simulink model "My_gfm_battery_sil_1_Exciter_Dis"  (R2018b)
settings: Solver=ode23t  StartTime=0.0  StopTime=5  MaxStep=1e-4  RelTol=1e-3
PreLoadFcn:
  | modelDir = fileparts(get_param(bdroot,'FileName'));
  | 
  | load_system(fullfile(modelDir,'controls_element_lib.slx'));
  | load_system(fullfile(modelDir,'test_sequence_lib.slx'));
InitFcn:
  | close all;
  | clear all;
  | clc;
  | 
  | % frequency nominals
  | F_NOM = 60;
  | W_NOM = 2 * pi * F_NOM;
  | 
  | % base values relative to inverter
  | % --------------------------------
  | VLL_INV_NOM = 480;
  | P_INV_NOM = 1e6;
  | Q_INV_NOM = 0.5e6;
  | S_INV_NOM = sqrt(P_INV_NOM^2 + Q_INV_NOM^2);
  | 
  | I_INV_BASE = S_INV_NOM/(sqrt(3)*VLL_INV_NOM);
  | Z_INV_BASE = VLL_INV_NOM^2/S_INV_NOM;
  | L_INV_BASE = Z_INV_BASE / W_NOM;
  | C_INV_BASE = 1 / (Z_INV_BASE * W_NOM);
  | 
  | % nominal ratings for power system model
  | % --------------------------------------
  | INVERTER_COUNT = 100;
  | 
  | VLV_NOM = VLL_INV_NOM;
  | VMV_NOM = 35e3;
  | VHV_NOM = 230e3;
  | S_PLANT = INVERTER_COUNT * S_INV_NOM;
  | 
  | N_GSU = VHV_NOM/VMV_NOM;
  | N_MVT = VMV_NOM/VLV_NOM;
  | 
  | I_LV_BASE = S_PLANT/(sqrt(3)*VLV_NOM);
  | I_MV_BASE = S_PLANT/(sqrt(3)*VMV_NOM);
  | I_HV_BASE = S_PLANT/(sqrt(3)*VHV_NOM);
  | 
  | Z_LV_BASE = VLV_NOM^2/S_PLANT;
  | Z_MV_BASE = VMV_NOM^2/S_PLANT;
  | Z_HV_BASE = VHV_NOM^2/S_PLANT;
  | 
  | L_LV_BASE = Z_LV_BASE / W_NOM;
  | L_MV_BASE = Z_MV_BASE / W_NOM;
  | L_HV_BASE = Z_HV_BASE / W_NOM;
  | C_LV_BASE = 1 / (Z_LV_BASE * W_NOM);
  | C_MV_BASE = 1 / (Z_MV_BASE * W_NOM);
  | C_HV_BASE = 1 / (Z_HV_BASE * W_NOM);
undefined symbols (not defined in the file): D1, D11, Delta, DiscIntNeverNeededParam, gcbh, j, sps_rtmsupport, Ts
libraries: powerlib x70, simulink x29, test_sequence_lib x10, controls_element_lib x3, spsHalfBridgeModel x3
(part 4 of 6)

== system My_gfm_battery_sil_1_Exciter_Dis/My Inverter Controller /My_acMonitor_A/Analyzer_V ==
  note: What is that?
  note: complex multiplication
  note: Let
      | V+*cos wt + V-*cos wt + vo * cos wt + vdc
      | V+*cos (wt-120) + V-*cos (wt+120) vo * cos wt + vdc
      | V+*cos (wt+120) + V-*cos (wt-120) vo * cos wt + vdc
  note: filter to remove pulsating on whatever
      | a frame coming from opposie rotating
  note: + conj
  note: Vd- , Vq-
  note: Vd+ , Vq+
  note: - conj
  note: Not sure why SOGI filter was not used
      | to get clean Pve and Nve
  note: cos x + j sin x
      | cos (x-120) + j (sin x -120)
      | cos (x+120) + j (sin x +120)
  note: cos x - j sin x
  note: V+/2*[1+cos2wt] + V-/2*[1+cos2wt] + vo/2*[1+cos2wt] + vdc * cos wt
      | V+/2*[cos(2pi/3)+cos(2wt-2pi/3)] + V-/2*[cos(2pi/3)+cos(2wt-4pi/3)] + vo/2*[1+cos2wt] + vdc * cos wt
      | V+/2*[cos(2pi/3)+cos(2wt-4pi/3)] + V-/2*[cos(2pi/3)+cos(2wt-2pi/3)] + vo/2*[1+cos2wt] + vdc * cos wt
      |
      | -V+/2*[sin2wt] - V-/2*[sin2wt] - vo/2*[sin2wt] - vdc * sin wt
      | -V+/2*[sin(2wt-2pi/3)+sin(2pi/3)] - V-/2*[sin(2wt-4pi/3)-sin(2pi/3)] - vo/2*[sin2wt] - vdc * sin wt
      | -V+/2*[sin(2wt-4pi/3)-sin(2pi/3)] - V-/2*[sin(2wt-2pi/3)+sin(2pi/3)] - vo/2*[sin2wt] - vdc * sin wt
  note: [ 1 ]
      | [ exp(- j2pi/3)]
      | [ exp(- j4pi/3)]
  note: [ 1 ]
      | [ exp(- j4pi/3)]
      | [ exp(- j8pi/3)] = [ exp(- j2pi/3)]
  note: Remove double frequency
      | V+/2+ V-/2+ vo/2 + vdc*coswt
      | V+/2*cos(2pi/3) + V-/2*cos(2pi/3) + vo/2 + vdc*coswt
      | V+/2*cos(2pi/3) + V-/2*cos(2pi/3) + vo/2 + vdc*coswt
      |
      | - vdc*sinwt
      | -V+/2*sin(2pi/3) - V-/2*-sin(2pi/3) - vdc*sinwt
      | -V+/2*-sin(2pi/3) - V-/2*+sin(2pi/3) - vdc*sinwt
  note: sqrt(2) *[V+/2+ V-/2+ vo/2 + vdc*coswt]
      | sqrt(2) *[V+/2*cos(2pi/3) + V-/2*cos(2pi/3) + vo/2 + vdc*coswt]
      | sqrt(2) *[V+/2*cos(2pi/3) + V-/2*cos(2pi/3) + vo/2 + vdc*coswt]
      |
      | sqrt(2) *[- vdc*sinwt]
      | sqrt(2) *[-V+/2*sin(2pi/3) - V-/2*-sin(2pi/3) - vdc*sinwt]
      | sqrt(2) *[-V+/2*-sin(2pi/3) - V-/2*+sin(2pi/3) - vdc*sinwt]
  note: 1
      | cos(-4pi/3)
      | cos(-2pi/3)
      |
      | 0
      | sin(-4pi/3)
      | sin(-2pi/3)
  note: 1
      | cos(-2pi/3)
      | cos(-4pi/3)
      |
      | 0
      | sin(-2pi/3)
      | sin(-4pi/3)
  note: sqrt(2) *[V+/2+ V-/2+ vo/2 + vdc*coswt] * 1 - sqrt(2) *[- vdc*sinwt] * 0
      | sqrt(2) *[V+/2*cos(2pi/3) + V-/2*cos(2pi/3) + vo/2 + vdc*coswt] * cos(-4pi/3) - sqrt(2) *[-V+/2*sin(2pi/3) - V-/2*-sin(2pi/3) - vdc*sinwt] * sin(-4pi/3)
      | sqrt(2) *[V+/2*cos(2pi/3) + V-/2*cos(2pi/3) + vo/2 + vdc*coswt] * cos(-2pi/3) - sqrt(2) *[-V+/2*-sin(2pi/3) - V-/2*+sin(2pi/3) - vdc*sinwt] * sin(-2pi/3)
      |
      | sqrt(2) *[V+/2+ V-/2+ vo/2 + vdc*coswt] * 0 + sqrt(2) *[- vdc*sinwt] * 1
      | sqrt(2) *[V+/2*cos(2pi/3) + V-/2*cos(2pi/3) + vo/2 + vdc*coswt] * sin(-4pi/3) + sqrt(2) *[-V+/2*sin(2pi/3) - V-/2*-sin(2pi/3) - vdc*sinwt] * cos(-4pi/3)
      | sqrt(2) *[V+/2*cos(2pi/3) + V-/2*cos(2pi/3) + vo/2 + vdc*coswt] * sin(-2pi/3) + sqrt(2) *[-V+/2*-sin(2pi/3) - V-/2*+sin(2pi/3) - vdc*sinwt] * cos(-2pi/3)
  note: 3 * sqrt(2) *[vo/2 + vdc*coswt]
      |
      | 3 * sqrt(2) *[- vdc*sinwt]
  note: sqrt(2) *[vo/2 + vdc*coswt]
      |
      | sqrt(2) *[- vdc*sinwt]
  note: sqrt(2) *[V+/2+ V-/2+ vo/2 + vdc*coswt]
      | sqrt(2) *[V+/2*-0.5 + V-/2*-0.5 + vo/2 + vdc*coswt] * -0.5 - sqrt(2) *[-V+/2*sqrt(3/2) - V-/2*-sqrt(3/2) - vdc*sinwt] * sqrt(3/2)
      | sqrt(2) *[V+/2*-0.5 + V-/2*-0.5 + vo/2 + vdc*coswt] * -0.5 - sqrt(2) *[-V+/2*-sqrt(3/2) - V-/2*+sqrt(3/2) - vdc*sinwt] * -sqrt(3/2)
      |
      | sqrt(2) *[V+/2+ V-/2+ vo/2 + vdc*coswt] * 0 + sqrt(2) *[- vdc*sinwt] * 1
      | sqrt(2) *[V+/2* -0.5 + V-/2* -0.5 + vo/2 + vdc*coswt] * sqrt(3/2) + sqrt(2) *[-V+/2* sqrt(3/2) - V-/2*- sqrt(3/2) - vdc*sinwt] * -0.5
      | sqrt(2) *[V+/2* -0.5 + V-/2* -0.5 + vo/2 + vdc*coswt] * - sqrt(3/2) + sqrt(2) *[-V+/2*- sqrt(3/2) - V-/2* sqrt(3/2) - vdc*sinwt] * -0.5
  note: sqrt(2) *[3 * V+/2+ 0 * V-/2+ 0 * vo/2 + 0 * vdc*coswt
      |
      | sqrt(2) *[0 * V+/2+ 0 * V-/2+ 0 * vo/2 + 0 * vdc*coswt
  note: sqrt(2) *[V+/2]
      |
      | 0
  note: sqrt(3) * sqrt(2) *[V+/2]
      |
      | 0
  note: sqrt(3) *sqrt(2) *[vo/2 + vdc*coswt]
      |
      | sqrt(3)* sqrt(2) *[- vdc*sinwt]
  note: sqrt(2) *[V+/2+ V-/2+ vo/2 + vdc*coswt] * 1 - sqrt(2) *[- vdc*sinwt] * 0
      | sqrt(2) *[V+/2*cos(2pi/3) + V-/2*cos(2pi/3) + vo/2 + vdc*coswt] * cos(-2pi/3) - sqrt(2) *[-V+/2*sin(2pi/3) - V-/2*-sin(2pi/3) - vdc*sinwt] * sin(-2pi/3)
      | sqrt(2) *[V+/2*cos(2pi/3) + V-/2*cos(2pi/3) + vo/2 + vdc*coswt] * cos(-4pi/3) - sqrt(2) *[-V+/2*-sin(2pi/3) - V-/2*+sin(2pi/3) - vdc*sinwt] * sin(-4pi/3)
      |
      | sqrt(2) *[V+/2+ V-/2+ vo/2 + vdc*coswt] * 0 + sqrt(2) *[- vdc*sinwt] * 1
      | sqrt(2) *[V+/2*cos(2pi/3) + V-/2*cos(2pi/3) + vo/2 + vdc*coswt] * sin(-2pi/3) + sqrt(2) *[-V+/2*sin(2pi/3) - V-/2*-sin(2pi/3) - vdc*sinwt] * cos(-2pi/3)
      | sqrt(2) *[V+/2*cos(2pi/3) + V-/2*cos(2pi/3) + vo/2 + vdc*coswt] * sin(-4pi/3) + sqrt(2) *[-V+/2*-sin(2pi/3) - V-/2*+sin(2pi/3) - vdc*sinwt] * cos(-4pi/3)
  note: sqrt(2) *[V+/2+ V-/2+ vo/2 + vdc*coswt]
      | sqrt(2) *[V+/2*-0.5 + V-/2*-0.5 + vo/2 + vdc*coswt] * -0.5 - sqrt(2) *[-V+/2*sqrt(3/2) - V-/2*-sqrt(3/2) - vdc*sinwt] * -sqrt(3/2)
      | sqrt(2) *[V+/2*-0.5 + V-/2*-0.5 + vo/2 + vdc*coswt] * -0.5 - sqrt(2) *[-V+/2*-sqrt(3/2) - V-/2*+sqrt(3/2) - vdc*sinwt] * sqrt(3/2)
      |
      | sqrt(2) *[V+/2+ V-/2+ vo/2 + vdc*coswt] * 0 + sqrt(2) *[- vdc*sinwt] * 1
      | sqrt(2) *[V+/2*-0.5 + V-/2*-0.5 + vo/2 + vdc*coswt] * -sqrt(3/2) + sqrt(2) *[-V+/2*sqrt(3/2) - V-/2*-sqrt(3/2) - vdc*sinwt] * -0.5
      | sqrt(2) *[V+/2*-0.5 + V-/2*-0.5 + vo/2 + vdc*coswt] * sqrt(3/2) + sqrt(2) *[-V+/2*-sqrt(3/2) - V-/2*sqrt(3/2) - vdc*sinwt] * -0.5
  note: sqrt(2) *[0 * V+/2+ 3 * V-/2+ 0 * vo/2 + 0 * vdc*coswt
      |
      | sqrt(2) *[0 * V+/2+ 0 * V-/2+ 0 * vo/2 + 0 * vdc*coswt
  note: sqrt(2) *[V-/2]
      |
      | 0
  note: sqrt(3) *sqrt(2) *[V-/2]
      |
      | 0
  note: sqrt(2) *[V+/2+ V-/2+ vo/2 + vdc*coswt]
      | sqrt(2) *[V+/2*cos(2pi/3) + V-/2*cos(2pi/3) + vo/2 + vdc*coswt] * cos(-4pi/3) - sqrt(2) *[-V+/2*sin(2pi/3) - V-/2*-sin(2pi/3) - vdc*sinwt] * sin(-4pi/3)
      | sqrt(2) *[V+/2*cos(2pi/3) + V-/2*cos(2pi/3) + vo/2 + vdc*coswt] * cos(-2pi/3) - sqrt(2) *[-V+/2*-sin(2pi/3) - V-/2*+sin(2pi/3) - vdc*sinwt] * sin(-2pi/3)
      |
      | sqrt(2) *[- vdc*sinwt]
      | sqrt(2) *[V+/2*cos(2pi/3) + V-/2*cos(2pi/3) + vo/2 + vdc*coswt] * sin(-4pi/3) + sqrt(2) *[-V+/2*sin(2pi/3) - V-/2*-sin(2pi/3) - vdc*sinwt] * cos(-4pi/3)
      | sqrt(2) *[V+/2*cos(2pi/3) + V-/2*cos(2pi/3) + vo/2 + vdc*coswt] * sin(-2pi/3) + sqrt(2) *[-V+/2*-sin(2pi/3) - V-/2*+sin(2pi/3) - vdc*sinwt] * cos(-2pi/3)
  in[3] : Inport
  osc[3] : Inport  Port=2
  Conj : Math  Operator=conj  SaturateOnIntegerOverflow=on
  Demux : Demux  Outputs=3
  Gain2 : Gain  Gain=1/3
  Gain3 : Gain  Gain=1/3
  Gain4 : Gain  Gain=1/3
  Gain5 : Gain  Gain=sqrt(2)
  Product1 : Product
  Product2 : Product
  Product3 : Product
  Rotation : Constant  Value=exp(j*2*pi*[0 -1/3 -2/3])
  Rotation1 : Constant  Value=exp(j*2*pi*[0 -1/3 -2/3])
  Square : Math  Operator=square  SaturateOnIntegerOverflow=on
  Sum of Elements1 : Sum  Inputs=+
  Sum of Elements2 : Sum  Inputs=+
  Sum of Elements3 : Sum  Inputs=+
  Terminator : Terminator
  Terminator1 : Terminator
  complex_LPF : Subsystem  mask{tau=0.05}
      mask prompts: tau "Time constant"
  convert_to_LL : Gain  Gain=sqrt(3)
  convert_to_LL1 : Gain  Gain=sqrt(3)
  convert_to_LL2 : Gain  Gain=sqrt(3)
  fund[3] : Outport  VectorParamsAs1DForOutWhenUnconnected=on
  Zero : Outport  Port=2  VectorParamsAs1DForOutWhenUnconnected=on
  Pve : Outport  Port=3  VectorParamsAs1DForOutWhenUnconnected=on
  Nve : Outport  Port=4  VectorParamsAs1DForOutWhenUnconnected=on
  wires:
  convert_to_LL2/1 -> Nve/1
  convert_to_LL1/1 -> Pve/1
  convert_to_LL/1 -> Zero/1
  Gain4/1 -> convert_to_LL2/1
  complex_LPF/1(Out1) -> Gain5/1
  Product3/1 -> Sum of Elements3/1
  Product1/1 -> complex_LPF/1(In1)
  Demux/1 -> Conj/1
  Rotation/1 -> Square/1
  Rotation1/1 -> Product3/2
  Sum of Elements2/1 -> Gain3/1
  Conj/1 -> Product1/2
  Sum of Elements1/1 -> Gain2/1
  Square/1 -> Product2/2
  Sum of Elements3/1 -> Gain4/1
  osc[3]/1 -> Demux/1
  Gain3/1 -> convert_to_LL1/1
  Gain2/1 -> convert_to_LL/1
  in[3]/1 -> Product1/1
  Demux/2 -> Terminator/1
  Demux/3 -> Terminator1/1
  Gain5/1 -> Sum of Elements1/1, Product3/1, Product2/1
  Product2/1 -> Sum of Elements2/1, fund[3]/1

== system My_gfm_battery_sil_1_Exciter_Dis/My Inverter Controller /My_acMonitor_A/Analyzer_V1 ==
  note: Let Va coswt, so
      | V/2 *[ exp(jw) +exp(-jw)]
      | V/2 *[ exp(jw - j2pi/3) +exp(-jw + j2pi/3)]
      | V/2 *[ exp(jw - j4pi/3) +exp(-jw + j4pi/3)]
  note: filter to remove pulsating on whatever
      | a frame coming from opposie rotating
  note: + conj
  note: Vd- , Vq-
  note: Vd+ , Vq+
  note: - conj
  note: Not sure why SOGI filter was not used
      | to get clean Pve and Nve
  note: cos x + j sin x
      | cos (x-120) + j (sin x -120)
      | cos (x+120) + j (sin x +120)
  note: cos x - j sin x
  note: V/2 *[ 1 +exp(-2jw)]
      | V/2 *[ exp(- j2pi/3) +exp(-2jw + j2pi/3)]
      | V/2 *[ exp(- j4pi/3) +exp(-2jw + j4pi/3)]
  note: Remove double frequency
      | V/2 *[ 1 ]
      | V/2 *[ exp(- j2pi/3)]
      | V/2 *[ exp(- j4pi/3)]
  note: sqrt(2) * V/2 *[ 1 ]
      | sqrt(2) * V/2 *[ exp(- j2pi/3)]
      | sqrt(2) * V/2 *[ exp(- j4pi/3)]
  note: [ 1 ]
      | [ exp(- j2pi/3)]
      | [ exp(- j4pi/3)]
  note: sqrt(2) * V/2 *[ 1 ]
      | sqrt(2) * V/2 *[ exp(- j4pi/3)]
      | sqrt(2) * V/2 *[ exp(- j8pi/3)] = sqrt(2) * V/2 *[ exp(- j2pi/3)]
  note: [ 1 ]
      | [ exp(- j4pi/3)]
      | [ exp(- j8pi/3)] = [ exp(- j2pi/3)]
  note: sqrt(2) * V/2 *[ 1 ]
      | sqrt(2) * V/2 *[ exp(- j6pi/3)] = sqrt(2) * Vb/2
      | sqrt(2) * V/2 *[ exp(- j6pi/3)] = sqrt(2) * Vc/2
  note: sqrt(2) * V/2 *[ 1 ]
      | + sqrt(2) * V/2 *[ exp(- j2pi/3)]
      | + sqrt(2) * V/2 *[ exp(- j4pi/3)]
      | = 0
  note: sqrt(2) * V/2
      | + sqrt(2) * V/2
      | + sqrt(2) * V/2
      | = 3 * sqrt(2) * V/2 * 1/3 = V/sqrt(2)
      | The LN RMS
  note: sqrt(2) * V/2
      | + sqrt(2) * V/2 *[ exp(- j4pi/3)]
      | + sqrt(2) * V/2 *[ exp(- j2pi/3)]
      | = 0
      | The LN RMS
  in[3] : Inport
  osc[3] : Inport  Port=2
  Conj : Math  Operator=conj  SaturateOnIntegerOverflow=on
  Demux : Demux  Outputs=3
  Gain2 : Gain  Gain=1/3
  Gain3 : Gain  Gain=1/3
  Gain4 : Gain  Gain=1/3
  Gain5 : Gain  Gain=sqrt(2)
  Product1 : Product
  Product2 : Product
  Product3 : Product
  Rotation : Constant  Value=exp(j*2*pi*[0 -1/3 -2/3])
  Rotation1 : Constant  Value=exp(j*2*pi*[0 -1/3 -2/3])
  Square : Math  Operator=square  SaturateOnIntegerOverflow=on
  Sum of Elements1 : Sum  Inputs=+
  Sum of Elements2 : Sum  Inputs=+
  Sum of Elements3 : Sum  Inputs=+
  Terminator : Terminator
  Terminator1 : Terminator
  complex_LPF : Subsystem  mask{tau=0.05}
      mask prompts: tau "Time constant"
  convert_to_LL : Gain  Gain=sqrt(3)
  convert_to_LL1 : Gain  Gain=sqrt(3)
  convert_to_LL2 : Gain  Gain=sqrt(3)
  fund[3] : Outport  VectorParamsAs1DForOutWhenUnconnected=on
  Zero : Outport  Port=2  VectorParamsAs1DForOutWhenUnconnected=on
  Pve : Outport  Port=3  VectorParamsAs1DForOutWhenUnconnected=on
  Nve : Outport  Port=4  VectorParamsAs1DForOutWhenUnconnected=on
  wires:
  convert_to_LL2/1 -> Nve/1
  convert_to_LL1/1 -> Pve/1
  convert_to_LL/1 -> Zero/1
  Gain4/1 -> convert_to_LL2/1
  Product2/1 -> fund[3]/1, Sum of Elements2/1
  complex_LPF/1(Out1) -> Gain5/1
  Product3/1 -> Sum of Elements3/1
  Product1/1 -> complex_LPF/1(In1)
  Demux/1 -> Conj/1
  Rotation/1 -> Square/1
  Rotation1/1 -> Product3/2
  Sum of Elements2/1 -> Gain3/1
  Conj/1 -> Product1/2
  Sum of Elements1/1 -> Gain2/1
  Square/1 -> Product2/2
  Sum of Elements3/1 -> Gain4/1
  osc[3]/1 -> Demux/1
  Gain3/1 -> convert_to_LL1/1
  Gain2/1 -> convert_to_LL/1
  in[3]/1 -> Product1/1
  Demux/2 -> Terminator/1
  Demux/3 -> Terminator1/1
  Gain5/1 -> Sum of Elements1/1, Product3/1, Product2/1

== system My_gfm_battery_sil_1_Exciter_Dis/My Inverter Controller /My_acMonitor_A/PLL_3ph ==
  note: cos x - j sin x
      | cos (x-120) - j (sin x -120)
      | cos (x+120) - j (sin x +120)
  note: cos x + j sin x
      | cos (x-120) + j (sin x -120)
      | cos (x+120) + j (sin x +120)
  note: -sin x
      |  -sin (x -120)
      |  -sin (x +120)
  note: Vq
  note: filter 120 Hz, due to negative sequence
  note: Leaky Integrator
  note: vd = Va * cos x + Vb * cos (x-120) + Vc * cos (x+120)
  note: vq = -Va * sin x - Vb * sin (x-120) - Vc * sin (x+120)
  note: Va = vd * cos x - vq * sin x
  note: Vb = vd * cos (x-120) - vq * sin (x-120)
  note: Vc = vd * cos (x+120) - vq * sin (x+120)
  ref : Inport
  Complex to Real-Imag : ComplexToRealImag
  Conj : Math  Operator=conj  SaturateOnIntegerOverflow=on
  Constant : Constant  Value=120
  Gain1 : Gain  Gain=1.5
  Gain2 : Gain  Gain=4.5
  Gain3 : Gain  Gain=10e-3
  Integrator : Integrator  LimitOutput=on  UpperSaturationLimit=5  LowerSaturationLimit=-5
  Product : Product
  SOGI : controls_element_lib/dcVoltageRegulator_A/SOGI  SystemSampleTime=-1
  Saturation : Saturate  UpperLimit=5  LowerLimit=-5
  Sum : Sum  Inputs=+++
  Sum of Elements : Sum  Inputs=+
  Sum1 : Sum  Inputs=|+-
  Terminator : Terminator
  Terminator1 : Terminator
  Transfer Fcn : TransferFcn  Denominator=[0.02 1]
  f_nom : Constant  Value=nominalFrequency
  oscillator_3ph : Subsystem
  osc[3] : Outport  VectorParamsAs1DForOutWhenUnconnected=on
  freq : Outport  Port=2  VectorParamsAs1DForOutWhenUnconnected=on
  wires:
  Constant/1 -> SOGI/2
  Transfer Fcn/1 -> SOGI/1  "phase_error"
  f_nom/1 -> Sum/1
  Gain3/1 -> Sum1/2
  Sum of Elements/1 -> Transfer Fcn/1
  SOGI/1 -> Gain1/1, Gain2/1  "phase_error"
  Saturation/1 -> Sum/2
  Product/1 -> Sum of Elements/1
  Sum/1 -> freq/1, oscillator_3ph/1(f)  "freq"
  oscillator_3ph/1(osc[3]) -> Conj/1, osc[3]/1
  Gain2/1 -> Sum1/1
  Complex to Real-Imag/2 -> Product/2
  Sum1/1 -> Integrator/1
  Integrator/1 -> Gain3/1, Sum/3
  ref/1 -> Product/1
  Conj/1 -> Complex to Real-Imag/1
  Gain1/1 -> Saturation/1
  Complex to Real-Imag/1 -> Terminator/1
  SOGI/2 -> Terminator1/1

== system My_gfm_battery_sil_1_Exciter_Dis/My Inverter Controller /My_acMonitor_A/RMS_Analyzer ==
  in : Inport
  Gain : Gain  Gain=2 * pi * 10
  Integrator : Integrator  InitialCondition=0.01
  Sqrt : Sqrt  SaturateOnIntegerOverflow=on
  Square : Math  Operator=square  SaturateOnIntegerOverflow=on
  Sum : Sum  Inputs=|+-
  RMS : Outport  VectorParamsAs1DForOutWhenUnconnected=on
  wires:
  Square/1 -> Sum/1
  in/1 -> Square/1
  Gain/1 -> Integrator/1
  Sum/1 -> Gain/1
  Integrator/1 -> Sum/2, Sqrt/1
  Sqrt/1 -> RMS/1

== system My_gfm_battery_sil_1_Exciter_Dis/My Inverter Controller /My_acMonitor_A/SOGI ==
  in : Inport
  fnom : Inport  Port=2
  2pi : Gain  Gain=2*pi
  Integrator2 : Integrator
  Integrator3 : Integrator
  Product : Product
  Product1 : Product
  Sum4 : Sum  Inputs=|+-
  Sum5 : Sum  Inputs=|+-
  alpha : Gain  Gain=1 / sqrt(2)
  notch : Outport  VectorParamsAs1DForOutWhenUnconnected=on
  bpf : Outport  Port=2  VectorParamsAs1DForOutWhenUnconnected=on
  wires:
  Product1/1 -> Integrator3/1
  Product/1 -> Integrator2/1
  2pi/1 -> Product/2, Product1/2
  Integrator3/1 -> Sum4/2
  Sum4/1 -> Product/1
  Sum5/1 -> notch/1, alpha/1
  alpha/1 -> Sum4/1
  Integrator2/1 -> bpf/1, Sum5/2, Product1/1
  fnom/1 -> 2pi/1
  in/1 -> Sum5/1

== system My_gfm_battery_sil_1_Exciter_Dis/My Inverter Controller /My_circuit_controls_A/LPF1 ==
  note: Forward integrator
  in : Inport
  Constant2 : Constant  Value=Ts
  Constant3 : Constant  Value=OmegaUp
  Constant4 : Constant  Value=OmegaDn
  Constant9 : Constant  Value=1/20000
  Delay : Delay  DelayLength=1  InitialCondition=0
  Gain : Gain  Gain=1/5
  Math Function : Math  Operator=reciprocal  SaturateOnIntegerOverflow=on
  MinMax : MinMax  Function=max  Inputs=2
  MinMax1 : MinMax  Inputs=2
  MinMax2 : MinMax  Inputs=2
  Product : Product
  Product1 : Product
  Product2 : Product
  Saturation : Saturate  UpperLimit=inf  LowerLimit=0
  Saturation1 : Saturate  UpperLimit=0  LowerLimit=-inf
  Sum : Sum  Inputs=|++
  Sum1 : Sum  Inputs=|++
  Sum4 : Sum  Inputs=|+-
  out : Outport  VectorParamsAs1DForOutWhenUnconnected=on
  wires:
  Delay/1 -> out/1, Sum4/2, Sum/2
  in/1 -> Sum4/1
  Sum4/1 -> Product2/1, Product1/2
  Sum/1 -> Delay/1
  Saturation/1 -> Sum1/1
  Saturation1/1 -> Sum1/2
  Sum1/1 -> Product/2
  Product/1 -> Sum/1
  [Ts] -> Product/1
  [OmegaUp] -> Product1/1
  [OmegaDn] -> Product2/2
  Constant2/1 -> MinMax/1
  MinMax/1 -> [Ts]
  Constant9/1 -> MinMax/2
  MinMax1/1 -> [OmegaUp]
  MinMax2/1 -> [OmegaDn]
  [Ts] -> Math Function/1
  Math Function/1 -> Gain/1
  Gain/1 -> MinMax1/2, MinMax2/1
  Constant3/1 -> MinMax1/1
  Constant4/1 -> MinMax2/2
  Product1/1 -> Saturation/1
  Product2/1 -> Saturation1/1

== system My_gfm_battery_sil_1_Exciter_Dis/My Inverter Controller /My_circuit_controls_A/LPF2 ==
  note: Forward integrator
  in : Inport
  Constant2 : Constant  Value=Ts
  Constant3 : Constant  Value=OmegaUp
  Constant4 : Constant  Value=OmegaDn
  Constant9 : Constant  Value=1/20000
  Delay : Delay  DelayLength=1  InitialCondition=0
  Gain : Gain  Gain=1/5
  Math Function : Math  Operator=reciprocal  SaturateOnIntegerOverflow=on
  MinMax : MinMax  Function=max  Inputs=2
  MinMax1 : MinMax  Inputs=2
  MinMax2 : MinMax  Inputs=2
  Product : Product
  Product1 : Product
  Product2 : Product
  Saturation : Saturate  UpperLimit=inf  LowerLimit=0
  Saturation1 : Saturate  UpperLimit=0  LowerLimit=-inf
  Sum : Sum  Inputs=|++
  Sum1 : Sum  Inputs=|++
  Sum4 : Sum  Inputs=|+-
  out : Outport  VectorParamsAs1DForOutWhenUnconnected=on
  wires:
  Delay/1 -> out/1, Sum4/2, Sum/2
  in/1 -> Sum4/1
  Sum4/1 -> Product2/1, Product1/2
  Sum/1 -> Delay/1
  Saturation/1 -> Sum1/1
  Saturation1/1 -> Sum1/2
  Sum1/1 -> Product/2
  Product/1 -> Sum/1
  [Ts] -> Product/1
  [OmegaUp] -> Product1/1
  [OmegaDn] -> Product2/2
  Constant2/1 -> MinMax/1
  MinMax/1 -> [Ts]
  Constant9/1 -> MinMax/2
  MinMax1/1 -> [OmegaUp]
  MinMax2/1 -> [OmegaDn]
  [Ts] -> Math Function/1
  Math Function/1 -> Gain/1
  Gain/1 -> MinMax1/2, MinMax2/1
  Constant3/1 -> MinMax1/1
  Constant4/1 -> MinMax2/2
  Product1/1 -> Saturation/1
  Product2/1 -> Saturation1/1

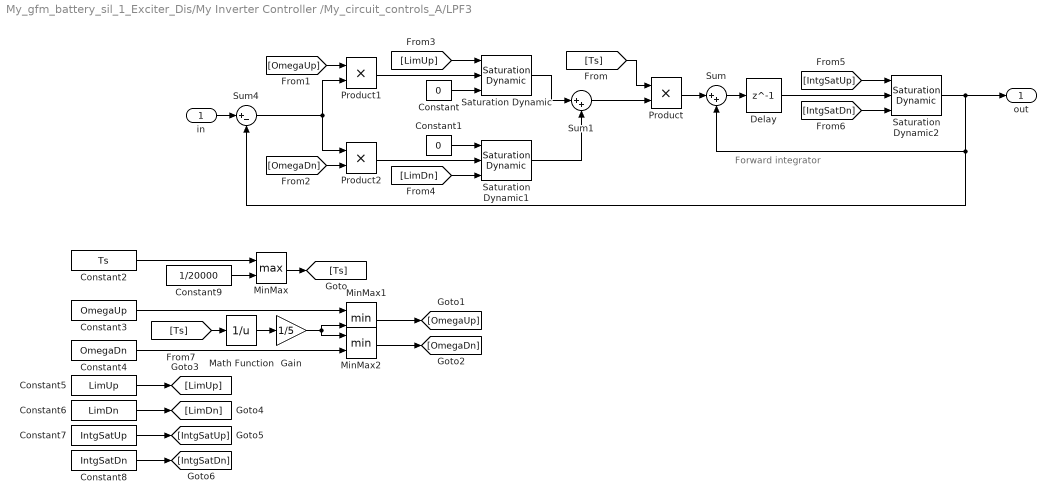
== system My_gfm_battery_sil_1_Exciter_Dis/My Inverter Controller /My_circuit_controls_A/LPF3 ==
  note: Forward integrator
  in : Inport
  Constant : Constant  Value=0
  Constant1 : Constant  Value=0
  Constant2 : Constant  Value=Ts
  Constant3 : Constant  Value=OmegaUp
  Constant4 : Constant  Value=OmegaDn
  Constant5 : Constant  Value=LimUp
  Constant6 : Constant  Value=LimDn
  Constant7 : Constant  Value=IntgSatUp
  Constant8 : Constant  Value=IntgSatDn
  Constant9 : Constant  Value=1/20000
  Delay : Delay  DelayLength=1  InitialCondition=0
  Gain : Gain  Gain=1/5
  Math Function : Math  Operator=reciprocal  SaturateOnIntegerOverflow=on
  MinMax : MinMax  Function=max  Inputs=2
  MinMax1 : MinMax  Inputs=2
  MinMax2 : MinMax  Inputs=2
  Product : Product
  Product1 : Product
  Product2 : Product
  Saturation Dynamic : simulink/Discontinuities/Saturation Dynamic  OutMin=[]  OutMax=[]  OutDataTypeStr=Inherit: Same as second input  OutDataType=fixdt(1, 16)  OutScaling=2^-10  DoSatur=off
  Saturation Dynamic1 : simulink/Discontinuities/Saturation Dynamic  OutMin=[]  OutMax=[]  OutDataTypeStr=Inherit: Same as second input  OutDataType=fixdt(1, 16)  OutScaling=2^-10  DoSatur=off
  Saturation Dynamic2 : simulink/Discontinuities/Saturation Dynamic  OutMin=[]  OutMax=[]  OutDataTypeStr=Inherit: Same as second input  OutDataType=fixdt(1, 16)  OutScaling=2^-10  DoSatur=off
  Sum : Sum  Inputs=|++
  Sum1 : Sum  Inputs=|++
  Sum4 : Sum  Inputs=|+-
  out : Outport  VectorParamsAs1DForOutWhenUnconnected=on
  wires:
  Saturation Dynamic2/1 -> Sum/2, Sum4/2, out/1
  in/1 -> Sum4/1
  Sum4/1 -> Product2/1, Product1/2
  Product1/1 -> Saturation Dynamic/2
  Product2/1 -> Saturation Dynamic1/2
  Sum/1 -> Delay/1
  Delay/1 -> Saturation Dynamic2/2
  Saturation Dynamic/1 -> Sum1/1
  Saturation Dynamic1/1 -> Sum1/2
  Sum1/1 -> Product/2
  Product/1 -> Sum/1
  [Ts] -> Product/1
  [OmegaUp] -> Product1/1
  [OmegaDn] -> Product2/2
  Constant/1 -> Saturation Dynamic/3
  Constant1/1 -> Saturation Dynamic1/1
  [LimUp] -> Saturation Dynamic/1
  [LimDn] -> Saturation Dynamic1/3
  Constant2/1 -> MinMax/1
  Constant5/1 -> [LimUp]
  Constant6/1 -> [LimDn]
  [IntgSatUp] -> Saturation Dynamic2/1
  [IntgSatDn] -> Saturation Dynamic2/3
  Constant7/1 -> [IntgSatUp]
  Constant8/1 -> [IntgSatDn]
  MinMax/1 -> [Ts]
  Constant9/1 -> MinMax/2
  MinMax1/1 -> [OmegaUp]
  MinMax2/1 -> [OmegaDn]
  [Ts] -> Math Function/1
  Math Function/1 -> Gain/1
  Gain/1 -> MinMax1/2, MinMax2/1
  Constant3/1 -> MinMax1/1
  Constant4/1 -> MinMax2/2

== system My_gfm_battery_sil_1_Exciter_Dis/My Inverter Controller /My_circuit_controls_A/LPF4 ==
  note: Forward integrator
  in : Inport
  Constant2 : Constant  Value=Ts
  Constant3 : Constant  Value=OmegaUp
  Constant4 : Constant  Value=OmegaDn
  Constant9 : Constant  Value=1/20000
  Delay : Delay  DelayLength=1  InitialCondition=0
  Gain : Gain  Gain=1/5
  Math Function : Math  Operator=reciprocal  SaturateOnIntegerOverflow=on
  MinMax : MinMax  Function=max  Inputs=2
  MinMax1 : MinMax  Inputs=2
  MinMax2 : MinMax  Inputs=2
  Product : Product
  Product1 : Product
  Product2 : Product
  Saturation : Saturate  UpperLimit=inf  LowerLimit=0
  Saturation1 : Saturate  UpperLimit=0  LowerLimit=-inf
  Sum : Sum  Inputs=|++
  Sum1 : Sum  Inputs=|++
  Sum4 : Sum  Inputs=|+-
  out : Outport  VectorParamsAs1DForOutWhenUnconnected=on
  wires:
  Delay/1 -> out/1, Sum4/2, Sum/2
  in/1 -> Sum4/1
  Sum4/1 -> Product2/1, Product1/2
  Sum/1 -> Delay/1
  Saturation/1 -> Sum1/1
  Saturation1/1 -> Sum1/2
  Sum1/1 -> Product/2
  Product/1 -> Sum/1
  [Ts] -> Product/1
  [OmegaUp] -> Product1/1
  [OmegaDn] -> Product2/2
  Constant2/1 -> MinMax/1
  MinMax/1 -> [Ts]
  Constant9/1 -> MinMax/2
  MinMax1/1 -> [OmegaUp]
  MinMax2/1 -> [OmegaDn]
  [Ts] -> Math Function/1
  Math Function/1 -> Gain/1
  Gain/1 -> MinMax1/2, MinMax2/1
  Constant3/1 -> MinMax1/1
  Constant4/1 -> MinMax2/2
  Product1/1 -> Saturation/1
  Product2/1 -> Saturation1/1

== system My_gfm_battery_sil_1_Exciter_Dis/My Inverter Controller /My_circuit_controls_A/LPF5 ==
  note: Forward integrator
  in : Inport
  Constant2 : Constant  Value=Ts
  Constant3 : Constant  Value=OmegaUp
  Constant4 : Constant  Value=OmegaDn
  Constant9 : Constant  Value=1/20000
  Delay : Delay  DelayLength=1  InitialCondition=0
  Gain : Gain  Gain=1/5
  Math Function : Math  Operator=reciprocal  SaturateOnIntegerOverflow=on
  MinMax : MinMax  Function=max  Inputs=2
  MinMax1 : MinMax  Inputs=2
  MinMax2 : MinMax  Inputs=2
  Product : Product
  Product1 : Product
  Product2 : Product
  Saturation : Saturate  UpperLimit=inf  LowerLimit=0
  Saturation1 : Saturate  UpperLimit=0  LowerLimit=-inf
  Sum : Sum  Inputs=|++
  Sum1 : Sum  Inputs=|++
  Sum4 : Sum  Inputs=|+-
  out : Outport  VectorParamsAs1DForOutWhenUnconnected=on
  wires:
  Delay/1 -> out/1, Sum4/2, Sum/2
  in/1 -> Sum4/1
  Sum4/1 -> Product2/1, Product1/2
  Sum/1 -> Delay/1
  Saturation/1 -> Sum1/1
  Saturation1/1 -> Sum1/2
  Sum1/1 -> Product/2
  Product/1 -> Sum/1
  [Ts] -> Product/1
  [OmegaUp] -> Product1/1
  [OmegaDn] -> Product2/2
  Constant2/1 -> MinMax/1
  MinMax/1 -> [Ts]
  Constant9/1 -> MinMax/2
  MinMax1/1 -> [OmegaUp]
  MinMax2/1 -> [OmegaDn]
  [Ts] -> Math Function/1
  Math Function/1 -> Gain/1
  Gain/1 -> MinMax1/2, MinMax2/1
  Constant3/1 -> MinMax1/1
  Constant4/1 -> MinMax2/2
  Product1/1 -> Saturation/1
  Product2/1 -> Saturation1/1

== system My_gfm_battery_sil_1_Exciter_Dis/My Inverter Controller /My_circuit_controls_A/SOGI ==
  in : Inport
  f : Inport  Port=2
  Constant2 : Constant  Value=Ts
  Constant9 : Constant  Value=1/20000
  Gain : Gain
  Gain2 : Gain  Gain=2*pi
  Integrator1 : Subsystem
  Integrator3 : Subsystem
  MinMax : MinMax  Function=max  Inputs=2
  Product : Product
  Product2 : Product
  Sum : Sum  Inputs=|+-
  Sum1 : Sum  Inputs=|+-
  Notched : Outport  VectorParamsAs1DForOutWhenUnconnected=on
  BandPassed : Outport  Port=2  VectorParamsAs1DForOutWhenUnconnected=on
  wires:
  f/1 -> Gain2/1
  in/1 -> Sum1/1
  Integrator1/1(Out) -> Product2/1
  Gain/1 -> Sum1/2
  Sum1/1 -> Notched/1, Sum/1
  Integrator3/1(Out) -> Gain/1, BandPassed/1, Integrator1/1(In)
  Gain2/1 -> Product2/2, Product/2
  Sum/1 -> Product/1
  Product2/1 -> Sum/2
  [Ts] -> Integrator3/2(Ts)
  Product/1 -> Integrator3/1(In)
  [Ts] -> Integrator1/2(Ts)
  MinMax/1 -> [Ts]
  Constant2/1 -> MinMax/1
  Constant9/1 -> MinMax/2

== system My_gfm_battery_sil_1_Exciter_Dis/My Inverter Controller /My_circuit_controls_A/SOGI_BPF1 ==
  in : Inport
  f : Inport  Port=2
  Gain : Gain
  Gain2 : Gain  Gain=2*pi
  Integrator : Integrator
  Integrator1 : Integrator
  Product : Product
  Product2 : Product
  Sum : Sum  Inputs=|+-
  Sum1 : Sum  Inputs=|+-
  Notched : Outport  VectorParamsAs1DForOutWhenUnconnected=on
  BandPassed : Outport  Port=2  VectorParamsAs1DForOutWhenUnconnected=on
  wires:
  f/1 -> Gain2/1
  in/1 -> Sum1/1
  Product/1 -> Integrator/1
  Integrator1/1 -> Product2/1
  Gain/1 -> Sum1/2
  Sum1/1 -> Notched/1, Sum/1
  Integrator/1 -> BandPassed/1, Integrator1/1, Gain/1
  Gain2/1 -> Product2/2, Product/2
  Sum/1 -> Product/1
  Product2/1 -> Sum/2

== system My_gfm_battery_sil_1_Exciter_Dis/My Inverter Controller /My_circuit_controls_A/virtual damper ==
  v : Inport
  Damping HPF : Subsystem  mask(High Pass Filter){Ts=1/20000, OmegaUp=1/250e-6, OmegaDn=1/250e-6}
      mask prompts: Ts "Tsample"; OmegaUp "Up Path Bandwidth"; OmegaDn "Down Path Bandwidth"
      mask help: Min. Tsample is 1/20000; Max. Omega is 0.2/Ts
      mask DialogControl Container2 Prompt: Parameters
  g_damp : Gain  Gain=1/(0.8*Z_INV_BASE)
  i_damp : Outport  VectorParamsAs1DForOutWhenUnconnected=on
  wires:
  g_damp/1 -> i_damp/1
  v/1 -> Damping HPF/1(in)
  Damping HPF/1(out) -> g_damp/1

== system My_gfm_battery_sil_1_Exciter_Dis/My Inverter Controller /My_circuit_controls_A/virtual damper1 ==
  v : Inport
  1/tau_damp : Gain  Gain=1/250e-6
  Integrator : Integrator
  Sum : Sum  Inputs=|+-
  g_damp : Gain  Gain=1/(0.8*Z_INV_BASE)
  i_damp : Outport  VectorParamsAs1DForOutWhenUnconnected=on
  wires:
  g_damp/1 -> i_damp/1
  Sum/1 -> g_damp/1, 1/tau_damp/1
  v/1 -> Sum/1
  1/tau_damp/1 -> Integrator/1
  Integrator/1 -> Sum/2

== system My_gfm_battery_sil_1_Exciter_Dis/My Inverter Controller /My_circuit_controls_A1/LPF ==
  1 : Inport
  Gain2 : Gain  Gain=1/20e-6
  Integrator : Integrator
  Sum4 : Sum  Inputs=|+-
  Out1 : Outport  VectorParamsAs1DForOutWhenUnconnected=on
  wires:
  Gain2/1 -> Integrator/1
  Integrator/1 -> Sum4/2, Out1/1
  1/1 -> Sum4/1
  Sum4/1 -> Gain2/1

== system My_gfm_battery_sil_1_Exciter_Dis/My Inverter Controller /My_circuit_controls_A1/LPF1 ==
  note: Forward integrator
  in : Inport
  Constant2 : Constant  Value=Ts
  Constant3 : Constant  Value=OmegaUp
  Constant4 : Constant  Value=OmegaDn
  Constant9 : Constant  Value=1/20000
  Delay : Delay  DelayLength=1  InitialCondition=0
  Gain : Gain  Gain=1/5
  Math Function : Math  Operator=reciprocal  SaturateOnIntegerOverflow=on
  MinMax : MinMax  Function=max  Inputs=2
  MinMax1 : MinMax  Inputs=2
  MinMax2 : MinMax  Inputs=2
  Product : Product
  Product1 : Product
  Product2 : Product
  Saturation : Saturate  UpperLimit=inf  LowerLimit=0
  Saturation1 : Saturate  UpperLimit=0  LowerLimit=-inf
  Sum : Sum  Inputs=|++
  Sum1 : Sum  Inputs=|++
  Sum4 : Sum  Inputs=|+-
  out : Outport  VectorParamsAs1DForOutWhenUnconnected=on
  wires:
  Delay/1 -> out/1, Sum4/2, Sum/2
  in/1 -> Sum4/1
  Sum4/1 -> Product2/1, Product1/2
  Sum/1 -> Delay/1
  Saturation/1 -> Sum1/1
  Saturation1/1 -> Sum1/2
  Sum1/1 -> Product/2
  Product/1 -> Sum/1
  [Ts] -> Product/1
  [OmegaUp] -> Product1/1
  [OmegaDn] -> Product2/2
  Constant2/1 -> MinMax/1
  MinMax/1 -> [Ts]
  Constant9/1 -> MinMax/2
  MinMax1/1 -> [OmegaUp]
  MinMax2/1 -> [OmegaDn]
  [Ts] -> Math Function/1
  Math Function/1 -> Gain/1
  Gain/1 -> MinMax1/2, MinMax2/1
  Constant3/1 -> MinMax1/1
  Constant4/1 -> MinMax2/2
  Product1/1 -> Saturation/1
  Product2/1 -> Saturation1/1

== system My_gfm_battery_sil_1_Exciter_Dis/My Inverter Controller /My_circuit_controls_A1/LPF2 ==
  1 : Inport
  Gain2 : Gain  Gain=1/20e-6
  Integrator : Integrator
  Sum4 : Sum  Inputs=|+-
  Out1 : Outport  VectorParamsAs1DForOutWhenUnconnected=on
  wires:
  Sum4/1 -> Gain2/1
  1/1 -> Sum4/1
  Integrator/1 -> Out1/1, Sum4/2
  Gain2/1 -> Integrator/1

== system My_gfm_battery_sil_1_Exciter_Dis/My Inverter Controller /My_circuit_controls_A1/LPF3 ==
  note: Forward integrator
  in : Inport
  Constant2 : Constant  Value=Ts
  Constant3 : Constant  Value=OmegaUp
  Constant4 : Constant  Value=OmegaDn
  Constant9 : Constant  Value=1/20000
  Delay : Delay  DelayLength=1  InitialCondition=0
  Gain : Gain  Gain=1/5
  Math Function : Math  Operator=reciprocal  SaturateOnIntegerOverflow=on
  MinMax : MinMax  Function=max  Inputs=2
  MinMax1 : MinMax  Inputs=2
  MinMax2 : MinMax  Inputs=2
  Product : Product
  Product1 : Product
  Product2 : Product
  Saturation : Saturate  UpperLimit=inf  LowerLimit=0
  Saturation1 : Saturate  UpperLimit=0  LowerLimit=-inf
  Sum : Sum  Inputs=|++
  Sum1 : Sum  Inputs=|++
  Sum4 : Sum  Inputs=|+-
  out : Outport  VectorParamsAs1DForOutWhenUnconnected=on
  wires:
  Delay/1 -> out/1, Sum4/2, Sum/2
  in/1 -> Sum4/1
  Sum4/1 -> Product2/1, Product1/2
  Sum/1 -> Delay/1
  Saturation/1 -> Sum1/1
  Saturation1/1 -> Sum1/2
  Sum1/1 -> Product/2
  Product/1 -> Sum/1
  [Ts] -> Product/1
  [OmegaUp] -> Product1/1
  [OmegaDn] -> Product2/2
  Constant2/1 -> MinMax/1
  MinMax/1 -> [Ts]
  Constant9/1 -> MinMax/2
  MinMax1/1 -> [OmegaUp]
  MinMax2/1 -> [OmegaDn]
  [Ts] -> Math Function/1
  Math Function/1 -> Gain/1
  Gain/1 -> MinMax1/2, MinMax2/1
  Constant3/1 -> MinMax1/1
  Constant4/1 -> MinMax2/2
  Product1/1 -> Saturation/1
  Product2/1 -> Saturation1/1

== system My_gfm_battery_sil_1_Exciter_Dis/My Inverter Controller /My_circuit_controls_A1/LPF4 ==
  note: Forward integrator
  in : Inport
  Constant2 : Constant  Value=Ts
  Constant3 : Constant  Value=OmegaUp
  Constant4 : Constant  Value=OmegaDn
  Constant9 : Constant  Value=1/20000
  Delay : Delay  DelayLength=1  InitialCondition=0
  Gain : Gain  Gain=1/5
  Math Function : Math  Operator=reciprocal  SaturateOnIntegerOverflow=on
  MinMax : MinMax  Function=max  Inputs=2
  MinMax1 : MinMax  Inputs=2
  MinMax2 : MinMax  Inputs=2
  Product : Product
  Product1 : Product
  Product2 : Product
  Saturation : Saturate  UpperLimit=inf  LowerLimit=0
  Saturation1 : Saturate  UpperLimit=0  LowerLimit=-inf
  Sum : Sum  Inputs=|++
  Sum1 : Sum  Inputs=|++
  Sum4 : Sum  Inputs=|+-
  out : Outport  VectorParamsAs1DForOutWhenUnconnected=on
  wires:
  Delay/1 -> out/1, Sum4/2, Sum/2
  in/1 -> Sum4/1
  Sum4/1 -> Product2/1, Product1/2
  Sum/1 -> Delay/1
  Saturation/1 -> Sum1/1
  Saturation1/1 -> Sum1/2
  Sum1/1 -> Product/2
  Product/1 -> Sum/1
  [Ts] -> Product/1
  [OmegaUp] -> Product1/1
  [OmegaDn] -> Product2/2
  Constant2/1 -> MinMax/1
  MinMax/1 -> [Ts]
  Constant9/1 -> MinMax/2
  MinMax1/1 -> [OmegaUp]
  MinMax2/1 -> [OmegaDn]
  [Ts] -> Math Function/1
  Math Function/1 -> Gain/1
  Gain/1 -> MinMax1/2, MinMax2/1
  Constant3/1 -> MinMax1/1
  Constant4/1 -> MinMax2/2
  Product1/1 -> Saturation/1
  Product2/1 -> Saturation1/1

== system My_gfm_battery_sil_1_Exciter_Dis/My Inverter Controller /My_circuit_controls_A1/SOGI ==
  in : Inport
  f : Inport  Port=2
  Constant2 : Constant  Value=Ts
  Constant9 : Constant  Value=1/20000
  Gain : Gain
  Gain2 : Gain  Gain=2*pi
  Integrator1 : Subsystem
  Integrator3 : Subsystem
  MinMax : MinMax  Function=max  Inputs=2
  Product : Product
  Product2 : Product
  Sum : Sum  Inputs=|+-
  Sum1 : Sum  Inputs=|+-
  Notched : Outport  VectorParamsAs1DForOutWhenUnconnected=on
  BandPassed : Outport  Port=2  VectorParamsAs1DForOutWhenUnconnected=on
  wires:
  f/1 -> Gain2/1
  in/1 -> Sum1/1
  Integrator1/1(Out) -> Product2/1
  Gain/1 -> Sum1/2
  Sum1/1 -> Notched/1, Sum/1
  Integrator3/1(Out) -> Gain/1, BandPassed/1, Integrator1/1(In)
  Gain2/1 -> Product2/2, Product/2
  Sum/1 -> Product/1
  Product2/1 -> Sum/2
  [Ts] -> Integrator3/2(Ts)
  Product/1 -> Integrator3/1(In)
  [Ts] -> Integrator1/2(Ts)
  MinMax/1 -> [Ts]
  Constant2/1 -> MinMax/1
  Constant9/1 -> MinMax/2

== system My_gfm_battery_sil_1_Exciter_Dis/My Inverter Controller /My_circuit_controls_A1/virtual damper ==
  v : Inport
  Damping HPF : Subsystem  mask(High Pass Filter){Ts=1/20000, OmegaUp=1/250e-6, OmegaDn=1/250e-6}
      mask prompts: Ts "Tsample"; OmegaUp "Up Path Bandwidth"; OmegaDn "Down Path Bandwidth"
      mask help: Min. Tsample is 1/20000; Max. Omega is 0.2/Ts
      mask DialogControl Container2 Prompt: Parameters
  g_damp : Gain  Gain=1/(0.8*Z_INV_BASE)
  i_damp : Outport  VectorParamsAs1DForOutWhenUnconnected=on
  wires:
  g_damp/1 -> i_damp/1
  v/1 -> Damping HPF/1(in)
  Damping HPF/1(out) -> g_damp/1

== system My_gfm_battery_sil_1_Exciter_Dis/My Inverter Controller /My_circuit_controls_A2/LPF ==
  1 : Inport
  Gain2 : Gain  Gain=1/20e-6
  Integrator : Integrator
  Sum4 : Sum  Inputs=|+-
  Out1 : Outport  VectorParamsAs1DForOutWhenUnconnected=on
  wires:
  Gain2/1 -> Integrator/1
  Integrator/1 -> Sum4/2, Out1/1
  1/1 -> Sum4/1
  Sum4/1 -> Gain2/1

== system My_gfm_battery_sil_1_Exciter_Dis/My Inverter Controller /My_circuit_controls_A2/LPF1 ==
  1 : Inport
  Gain2 : Gain  Gain=1/20e-6
  Integrator : Integrator
  Sum4 : Sum  Inputs=|+-
  Out1 : Outport  VectorParamsAs1DForOutWhenUnconnected=on
  wires:
  Gain2/1 -> Integrator/1
  Integrator/1 -> Sum4/2, Out1/1
  1/1 -> Sum4/1
  Sum4/1 -> Gain2/1

== system My_gfm_battery_sil_1_Exciter_Dis/My Inverter Controller /My_circuit_controls_A2/LPF2 ==
  1 : Inport
  Gain2 : Gain  Gain=1/20e-6
  Integrator : Integrator
  Sum4 : Sum  Inputs=|+-
  Out1 : Outport  VectorParamsAs1DForOutWhenUnconnected=on
  wires:
  Sum4/1 -> Gain2/1
  1/1 -> Sum4/1
  Integrator/1 -> Out1/1, Sum4/2
  Gain2/1 -> Integrator/1

== system My_gfm_battery_sil_1_Exciter_Dis/My Inverter Controller /My_circuit_controls_A2/LPF3 ==
  1 : Inport
  Discrete-Time Integrator : DiscreteIntegrator  SampleTime=1/20000  ICPrevOutput=DiscIntNeverNeededParam  ICPrevScaledInput=DiscIntNeverNeededParam
  Gain2 : Gain  Gain=1/500e-6
  Sum4 : Sum  Inputs=|+-
  Out1 : Outport  VectorParamsAs1DForOutWhenUnconnected=on
  wires:
  Gain2/1 -> Discrete-Time Integrator/1
  Discrete-Time Integrator/1 -> Sum4/2, Out1/1
  1/1 -> Sum4/1
  Sum4/1 -> Gain2/1

== system My_gfm_battery_sil_1_Exciter_Dis/My Inverter Controller /My_circuit_controls_A2/LPF4 ==
  1 : Inport
  Discrete-Time Integrator : DiscreteIntegrator  SampleTime=1/20000  ICPrevOutput=DiscIntNeverNeededParam  ICPrevScaledInput=DiscIntNeverNeededParam
  Gain2 : Gain  Gain=1/500e-6
  Sum4 : Sum  Inputs=|+-
  Out1 : Outport  VectorParamsAs1DForOutWhenUnconnected=on
  wires:
  Gain2/1 -> Discrete-Time Integrator/1
  Discrete-Time Integrator/1 -> Sum4/2, Out1/1
  1/1 -> Sum4/1
  Sum4/1 -> Gain2/1

== system My_gfm_battery_sil_1_Exciter_Dis/My Inverter Controller /My_circuit_controls_A2/SOGI_BPF ==
  in : Inport
  f : Inport  Port=2
  Discrete-Time Integrator : DiscreteIntegrator  SampleTime=1/20000  ICPrevOutput=DiscIntNeverNeededParam  ICPrevScaledInput=DiscIntNeverNeededParam
  Discrete-Time Integrator1 : DiscreteIntegrator  SampleTime=1/20000  ICPrevOutput=DiscIntNeverNeededParam  ICPrevScaledInput=DiscIntNeverNeededParam
  Gain : Gain
  Gain2 : Gain  Gain=2*pi
  Product : Product
  Product2 : Product
  Sum : Sum  Inputs=|+-
  Sum1 : Sum  Inputs=|+-
  Notched : Outport  VectorParamsAs1DForOutWhenUnconnected=on
  wires:
  f/1 -> Gain2/1
  in/1 -> Sum1/1
  Product/1 -> Discrete-Time Integrator/1
  Gain/1 -> Sum1/2
  Sum1/1 -> Notched/1, Sum/1
  Gain2/1 -> Product2/2, Product/2
  Sum/1 -> Product/1
  Product2/1 -> Sum/2
  Discrete-Time Integrator/1 -> Discrete-Time Integrator1/1, Gain/1
  Discrete-Time Integrator1/1 -> Product2/1

== system My_gfm_battery_sil_1_Exciter_Dis/My Inverter Controller /My_circuit_controls_A2/virtual damper ==
  v : Inport
  1/tau_damp : Gain  Gain=1/250e-6
  Discrete-Time Integrator : DiscreteIntegrator  SampleTime=1/20000  ICPrevOutput=DiscIntNeverNeededParam  ICPrevScaledInput=DiscIntNeverNeededParam
  Sum : Sum  Inputs=|+-
  g_damp : Gain  Gain=1/(0.8*Z_INV_BASE)
  i_damp : Outport  VectorParamsAs1DForOutWhenUnconnected=on
  wires:
  g_damp/1 -> i_damp/1
  Sum/1 -> g_damp/1, 1/tau_damp/1
  v/1 -> Sum/1
  1/tau_damp/1 -> Discrete-Time Integrator/1
  Discrete-Time Integrator/1 -> Sum/2

== system My_gfm_battery_sil_1_Exciter_Dis/My Inverter Controller /My_circuit_controls_A3/LPF ==
  1 : Inport
  Gain2 : Gain  Gain=1/20e-6
  Integrator : Integrator
  Sum4 : Sum  Inputs=|+-
  Out1 : Outport  VectorParamsAs1DForOutWhenUnconnected=on
  wires:
  Gain2/1 -> Integrator/1
  Integrator/1 -> Sum4/2, Out1/1
  1/1 -> Sum4/1
  Sum4/1 -> Gain2/1

== system My_gfm_battery_sil_1_Exciter_Dis/My Inverter Controller /My_circuit_controls_A3/LPF1 ==
  1 : Inport
  Gain2 : Gain  Gain=1/20e-6
  Integrator : Integrator
  Sum4 : Sum  Inputs=|+-
  Out1 : Outport  VectorParamsAs1DForOutWhenUnconnected=on
  wires:
  Gain2/1 -> Integrator/1
  Integrator/1 -> Sum4/2, Out1/1
  1/1 -> Sum4/1
  Sum4/1 -> Gain2/1

== system My_gfm_battery_sil_1_Exciter_Dis/My Inverter Controller /My_circuit_controls_A3/LPF2 ==
  1 : Inport
  Gain2 : Gain  Gain=1/20e-6
  Integrator : Integrator
  Sum4 : Sum  Inputs=|+-
  Out1 : Outport  VectorParamsAs1DForOutWhenUnconnected=on
  wires:
  Sum4/1 -> Gain2/1
  1/1 -> Sum4/1
  Integrator/1 -> Out1/1, Sum4/2
  Gain2/1 -> Integrator/1

== system My_gfm_battery_sil_1_Exciter_Dis/My Inverter Controller /My_circuit_controls_A3/LPF3 ==
  note: Forward integrator
  in : Inport
  Constant2 : Constant  Value=Ts
  Constant3 : Constant  Value=OmegaUp
  Constant4 : Constant  Value=OmegaDn
  Constant9 : Constant  Value=1/20000
  Delay : Delay  DelayLength=1  InitialCondition=0
  Gain : Gain  Gain=1/5
  Math Function : Math  Operator=reciprocal  SaturateOnIntegerOverflow=on
  MinMax : MinMax  Function=max  Inputs=2
  MinMax1 : MinMax  Inputs=2
  MinMax2 : MinMax  Inputs=2
  Product : Product
  Product1 : Product
  Product2 : Product
  Saturation : Saturate  UpperLimit=inf  LowerLimit=0
  Saturation1 : Saturate  UpperLimit=0  LowerLimit=-inf
  Sum : Sum  Inputs=|++
  Sum1 : Sum  Inputs=|++
  Sum4 : Sum  Inputs=|+-
  out : Outport  VectorParamsAs1DForOutWhenUnconnected=on
  wires:
  Delay/1 -> out/1, Sum4/2, Sum/2
  in/1 -> Sum4/1
  Sum4/1 -> Product2/1, Product1/2
  Sum/1 -> Delay/1
  Saturation/1 -> Sum1/1
  Saturation1/1 -> Sum1/2
  Sum1/1 -> Product/2
  Product/1 -> Sum/1
  [Ts] -> Product/1
  [OmegaUp] -> Product1/1
  [OmegaDn] -> Product2/2
  Constant2/1 -> MinMax/1
  MinMax/1 -> [Ts]
  Constant9/1 -> MinMax/2
  MinMax1/1 -> [OmegaUp]
  MinMax2/1 -> [OmegaDn]
  [Ts] -> Math Function/1
  Math Function/1 -> Gain/1
  Gain/1 -> MinMax1/2, MinMax2/1
  Constant3/1 -> MinMax1/1
  Constant4/1 -> MinMax2/2
  Product1/1 -> Saturation/1
  Product2/1 -> Saturation1/1

== system My_gfm_battery_sil_1_Exciter_Dis/My Inverter Controller /My_circuit_controls_A3/LPF4 ==
  note: Forward integrator
  in : Inport
  Constant2 : Constant  Value=Ts
  Constant3 : Constant  Value=OmegaUp
  Constant4 : Constant  Value=OmegaDn
  Constant9 : Constant  Value=1/20000
  Delay : Delay  DelayLength=1  InitialCondition=0
  Gain : Gain  Gain=1/5
  Math Function : Math  Operator=reciprocal  SaturateOnIntegerOverflow=on
  MinMax : MinMax  Function=max  Inputs=2
  MinMax1 : MinMax  Inputs=2
  MinMax2 : MinMax  Inputs=2
  Product : Product
  Product1 : Product
  Product2 : Product
  Saturation : Saturate  UpperLimit=inf  LowerLimit=0
  Saturation1 : Saturate  UpperLimit=0  LowerLimit=-inf
  Sum : Sum  Inputs=|++
  Sum1 : Sum  Inputs=|++
  Sum4 : Sum  Inputs=|+-
  out : Outport  VectorParamsAs1DForOutWhenUnconnected=on
  wires:
  Delay/1 -> out/1, Sum4/2, Sum/2
  in/1 -> Sum4/1
  Sum4/1 -> Product2/1, Product1/2
  Sum/1 -> Delay/1
  Saturation/1 -> Sum1/1
  Saturation1/1 -> Sum1/2
  Sum1/1 -> Product/2
  Product/1 -> Sum/1
  [Ts] -> Product/1
  [OmegaUp] -> Product1/1
  [OmegaDn] -> Product2/2
  Constant2/1 -> MinMax/1
  MinMax/1 -> [Ts]
  Constant9/1 -> MinMax/2
  MinMax1/1 -> [OmegaUp]
  MinMax2/1 -> [OmegaDn]
  [Ts] -> Math Function/1
  Math Function/1 -> Gain/1
  Gain/1 -> MinMax1/2, MinMax2/1
  Constant3/1 -> MinMax1/1
  Constant4/1 -> MinMax2/2
  Product1/1 -> Saturation/1
  Product2/1 -> Saturation1/1

== system My_gfm_battery_sil_1_Exciter_Dis/My Inverter Controller /My_circuit_controls_A3/SOGI_BPF ==
  in : Inport
  f : Inport  Port=2
  Discrete-Time Integrator : DiscreteIntegrator  SampleTime=1/20000  ICPrevOutput=DiscIntNeverNeededParam  ICPrevScaledInput=DiscIntNeverNeededParam
  Discrete-Time Integrator1 : DiscreteIntegrator  SampleTime=1/20000  ICPrevOutput=DiscIntNeverNeededParam  ICPrevScaledInput=DiscIntNeverNeededParam
  Gain : Gain
  Gain2 : Gain  Gain=2*pi
  Product : Product
  Product2 : Product
  Sum : Sum  Inputs=|+-
  Sum1 : Sum  Inputs=|+-
  Notched : Outport  VectorParamsAs1DForOutWhenUnconnected=on
  wires:
  f/1 -> Gain2/1
  in/1 -> Sum1/1
  Product/1 -> Discrete-Time Integrator/1
  Discrete-Time Integrator/1 -> Discrete-Time Integrator1/1, Gain/1
  Gain/1 -> Sum1/2
  Sum1/1 -> Notched/1, Sum/1
  Gain2/1 -> Product2/2, Product/2
  Sum/1 -> Product/1
  Product2/1 -> Sum/2
  Discrete-Time Integrator1/1 -> Product2/1

== system My_gfm_battery_sil_1_Exciter_Dis/My Inverter Controller /My_circuit_controls_A3/virtual damper ==
  v : Inport
  Damping HPF : Subsystem  mask(High Pass Filter){Ts=1/20000, OmegaUp=1/250e-6, OmegaDn=1/250e-6}
      mask prompts: Ts "Tsample"; OmegaUp "Up Path Bandwidth"; OmegaDn "Down Path Bandwidth"
      mask help: Min. Tsample is 1/20000; Max. Omega is 0.2/Ts
      mask DialogControl Container2 Prompt: Parameters
  g_damp : Gain  Gain=1/(0.8*Z_INV_BASE)
  i_damp : Outport  VectorParamsAs1DForOutWhenUnconnected=on
  wires:
  g_damp/1 -> i_damp/1
  v/1 -> Damping HPF/1(in)
  Damping HPF/1(out) -> g_damp/1

== system My_gfm_battery_sil_1_Exciter_Dis/My Inverter Controller /My_circuit_controls_A4/LPF ==
  1 : Inport
  Gain2 : Gain  Gain=1/20e-6
  Integrator : Integrator
  Sum4 : Sum  Inputs=|+-
  Out1 : Outport  VectorParamsAs1DForOutWhenUnconnected=on
  wires:
  Gain2/1 -> Integrator/1
  Integrator/1 -> Sum4/2, Out1/1
  1/1 -> Sum4/1
  Sum4/1 -> Gain2/1

== system My_gfm_battery_sil_1_Exciter_Dis/My Inverter Controller /My_circuit_controls_A4/LPF1 ==
  note: Forward integrator
  in : Inport
  Constant2 : Constant  Value=Ts
  Constant3 : Constant  Value=OmegaUp
  Constant4 : Constant  Value=OmegaDn
  Constant9 : Constant  Value=1/20000
  Delay : Delay  DelayLength=1  InitialCondition=0
  Gain : Gain  Gain=1/5
  Math Function : Math  Operator=reciprocal  SaturateOnIntegerOverflow=on
  MinMax : MinMax  Function=max  Inputs=2
  MinMax1 : MinMax  Inputs=2
  MinMax2 : MinMax  Inputs=2
  Product : Product
  Product1 : Product
  Product2 : Product
  Saturation : Saturate  UpperLimit=inf  LowerLimit=0
  Saturation1 : Saturate  UpperLimit=0  LowerLimit=-inf
  Sum : Sum  Inputs=|++
  Sum1 : Sum  Inputs=|++
  Sum4 : Sum  Inputs=|+-
  out : Outport  VectorParamsAs1DForOutWhenUnconnected=on
  wires:
  Delay/1 -> out/1, Sum4/2, Sum/2
  in/1 -> Sum4/1
  Sum4/1 -> Product2/1, Product1/2
  Sum/1 -> Delay/1
  Saturation/1 -> Sum1/1
  Saturation1/1 -> Sum1/2
  Sum1/1 -> Product/2
  Product/1 -> Sum/1
  [Ts] -> Product/1
  [OmegaUp] -> Product1/1
  [OmegaDn] -> Product2/2
  Constant2/1 -> MinMax/1
  MinMax/1 -> [Ts]
  Constant9/1 -> MinMax/2
  MinMax1/1 -> [OmegaUp]
  MinMax2/1 -> [OmegaDn]
  [Ts] -> Math Function/1
  Math Function/1 -> Gain/1
  Gain/1 -> MinMax1/2, MinMax2/1
  Constant3/1 -> MinMax1/1
  Constant4/1 -> MinMax2/2
  Product1/1 -> Saturation/1
  Product2/1 -> Saturation1/1

== system My_gfm_battery_sil_1_Exciter_Dis/My Inverter Controller /My_circuit_controls_A4/LPF2 ==
  1 : Inport
  Gain2 : Gain  Gain=1/20e-6
  Integrator : Integrator
  Sum4 : Sum  Inputs=|+-
  Out1 : Outport  VectorParamsAs1DForOutWhenUnconnected=on
  wires:
  Sum4/1 -> Gain2/1
  1/1 -> Sum4/1
  Integrator/1 -> Out1/1, Sum4/2
  Gain2/1 -> Integrator/1

== system My_gfm_battery_sil_1_Exciter_Dis/My Inverter Controller /My_circuit_controls_A4/LPF3 ==
  note: Forward integrator
  in : Inport
  Constant2 : Constant  Value=Ts
  Constant3 : Constant  Value=OmegaUp
  Constant4 : Constant  Value=OmegaDn
  Constant9 : Constant  Value=1/20000
  Delay : Delay  DelayLength=1  InitialCondition=0
  Gain : Gain  Gain=1/5
  Math Function : Math  Operator=reciprocal  SaturateOnIntegerOverflow=on
  MinMax : MinMax  Function=max  Inputs=2
  MinMax1 : MinMax  Inputs=2
  MinMax2 : MinMax  Inputs=2
  Product : Product
  Product1 : Product
  Product2 : Product
  Saturation : Saturate  UpperLimit=inf  LowerLimit=0
  Saturation1 : Saturate  UpperLimit=0  LowerLimit=-inf
  Sum : Sum  Inputs=|++
  Sum1 : Sum  Inputs=|++
  Sum4 : Sum  Inputs=|+-
  out : Outport  VectorParamsAs1DForOutWhenUnconnected=on
  wires:
  Delay/1 -> out/1, Sum4/2, Sum/2
  in/1 -> Sum4/1
  Sum4/1 -> Product2/1, Product1/2
  Sum/1 -> Delay/1
  Saturation/1 -> Sum1/1
  Saturation1/1 -> Sum1/2
  Sum1/1 -> Product/2
  Product/1 -> Sum/1
  [Ts] -> Product/1
  [OmegaUp] -> Product1/1
  [OmegaDn] -> Product2/2
  Constant2/1 -> MinMax/1
  MinMax/1 -> [Ts]
  Constant9/1 -> MinMax/2
  MinMax1/1 -> [OmegaUp]
  MinMax2/1 -> [OmegaDn]
  [Ts] -> Math Function/1
  Math Function/1 -> Gain/1
  Gain/1 -> MinMax1/2, MinMax2/1
  Constant3/1 -> MinMax1/1
  Constant4/1 -> MinMax2/2
  Product1/1 -> Saturation/1
  Product2/1 -> Saturation1/1

== system My_gfm_battery_sil_1_Exciter_Dis/My Inverter Controller /My_circuit_controls_A4/LPF4 ==
  note: Forward integrator
  in : Inport
  Constant2 : Constant  Value=Ts
  Constant3 : Constant  Value=OmegaUp
  Constant4 : Constant  Value=OmegaDn
  Constant9 : Constant  Value=1/20000
  Delay : Delay  DelayLength=1  InitialCondition=0
  Gain : Gain  Gain=1/5
  Math Function : Math  Operator=reciprocal  SaturateOnIntegerOverflow=on
  MinMax : MinMax  Function=max  Inputs=2
  MinMax1 : MinMax  Inputs=2
  MinMax2 : MinMax  Inputs=2
  Product : Product
  Product1 : Product
  Product2 : Product
  Saturation : Saturate  UpperLimit=inf  LowerLimit=0
  Saturation1 : Saturate  UpperLimit=0  LowerLimit=-inf
  Sum : Sum  Inputs=|++
  Sum1 : Sum  Inputs=|++
  Sum4 : Sum  Inputs=|+-
  out : Outport  VectorParamsAs1DForOutWhenUnconnected=on
  wires:
  Delay/1 -> out/1, Sum4/2, Sum/2
  in/1 -> Sum4/1
  Sum4/1 -> Product2/1, Product1/2
  Sum/1 -> Delay/1
  Saturation/1 -> Sum1/1
  Saturation1/1 -> Sum1/2
  Sum1/1 -> Product/2
  Product/1 -> Sum/1
  [Ts] -> Product/1
  [OmegaUp] -> Product1/1
  [OmegaDn] -> Product2/2
  Constant2/1 -> MinMax/1
  MinMax/1 -> [Ts]
  Constant9/1 -> MinMax/2
  MinMax1/1 -> [OmegaUp]
  MinMax2/1 -> [OmegaDn]
  [Ts] -> Math Function/1
  Math Function/1 -> Gain/1
  Gain/1 -> MinMax1/2, MinMax2/1
  Constant3/1 -> MinMax1/1
  Constant4/1 -> MinMax2/2
  Product1/1 -> Saturation/1
  Product2/1 -> Saturation1/1

== system My_gfm_battery_sil_1_Exciter_Dis/My Inverter Controller /My_circuit_controls_A4/LPF5 ==
  1 : Inport
  Gain2 : Gain  Gain=1/20e-6
  Integrator : Integrator
  Sum4 : Sum  Inputs=|+-
  Out1 : Outport  VectorParamsAs1DForOutWhenUnconnected=on
  wires:
  Sum4/1 -> Gain2/1
  1/1 -> Sum4/1
  Integrator/1 -> Out1/1, Sum4/2
  Gain2/1 -> Integrator/1

== system My_gfm_battery_sil_1_Exciter_Dis/My Inverter Controller /My_circuit_controls_A4/SOGI ==
  in : Inport
  f : Inport  Port=2
  Constant2 : Constant  Value=Ts
  Constant9 : Constant  Value=1/20000
  Gain : Gain
  Gain2 : Gain  Gain=2*pi
  Integrator1 : Subsystem
  Integrator3 : Subsystem
  MinMax : MinMax  Function=max  Inputs=2
  Product : Product
  Product2 : Product
  Sum : Sum  Inputs=|+-
  Sum1 : Sum  Inputs=|+-
  Notched : Outport  VectorParamsAs1DForOutWhenUnconnected=on
  BandPassed : Outport  Port=2  VectorParamsAs1DForOutWhenUnconnected=on
  wires:
  f/1 -> Gain2/1
  in/1 -> Sum1/1
  Integrator1/1(Out) -> Product2/1
  Gain/1 -> Sum1/2
  Sum1/1 -> Notched/1, Sum/1
  Integrator3/1(Out) -> Gain/1, BandPassed/1, Integrator1/1(In)
  Gain2/1 -> Product2/2, Product/2
  Sum/1 -> Product/1
  Product2/1 -> Sum/2
  [Ts] -> Integrator3/2(Ts)
  Product/1 -> Integrator3/1(In)
  [Ts] -> Integrator1/2(Ts)
  MinMax/1 -> [Ts]
  Constant2/1 -> MinMax/1
  Constant9/1 -> MinMax/2
